simulink model "H08_MRR"  (R2026a)
settings: Solver=VariableStepAuto  StopTime=25  MaxStep=tau/25
InitFcn:
  | % Rendszerparaméterek
  | K = 1;
  | tau = 1;
  | xi = 2;
  | 
  | % Kezdeti értékek
  | y_0 = 0;
  | z_0 = 0;
settings Model: Creator=Szalay  LastModifiedBy=Szalay

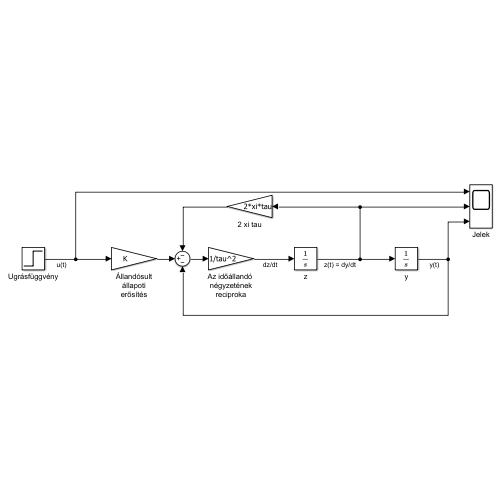
[thumbnail: Simulink's stored preview of the top-level diagram]
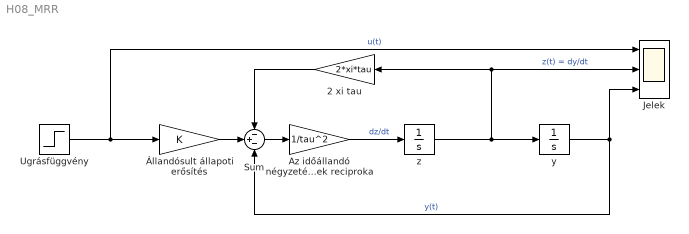
== system H08_MRR ==
  2 xi tau : Gain  Gain=2*xi*tau
  Az időállandó négyzetének reciproka : Gain  Gain=1/tau^2
  Jelek : Scope  NumInputPorts=3
      settings: ActiveDisplayYMinimum=-0.12499999999999997  ActiveDisplayYMaximum=1.125
  Sum : Sum  Inputs=-+-
  Ugrásfüggvény : Step  SampleTime=0
  y : Integrator  InitialCondition=y_0
  z : Integrator  InitialCondition=z_0
  Állandósult állapoti erősítés : Gain  Gain=K
  wires:
  z/1 -> Jelek/2, 2 xi tau/1, y/1  "z(t) = dy/dt"
  y/1 -> Jelek/3, Sum/3  "y(t)"
  Az időállandó négyzetének reciproka/1 -> z/1  "dz/dt"
  Sum/1 -> Az időállandó négyzetének reciproka/1
  Állandósult állapoti erősítés/1 -> Sum/2
  Ugrásfüggvény/1 -> Jelek/1, Állandósult állapoti erősítés/1  "u(t)"
  2 xi tau/1 -> Sum/1
